simulink model "mpc_ttype_psm"  (R2026a)
settings: Solver=ode23tb  StopTime=param.sim.simlength  FixedStep=param.glb_time.tc  MaxStep=param.glb_time.tc
values from neighbouring files (symbols this model uses):
  param = struct()    [init_model.m]
libraries: fl_lib x25, nesl_utility x12, cstblocks_lti x6, lithium_ion_battery x1, dclink_for_three_levels x1, three_phase_three_level_ttype_inverter_ideal_switch_based_model x1, single_phase_pwm_modulator x1, threephase_inductor_lib x1, simple_flexible_shaft x1, permanent_magnet_synchronous_machine x1
(part 3 of 4)

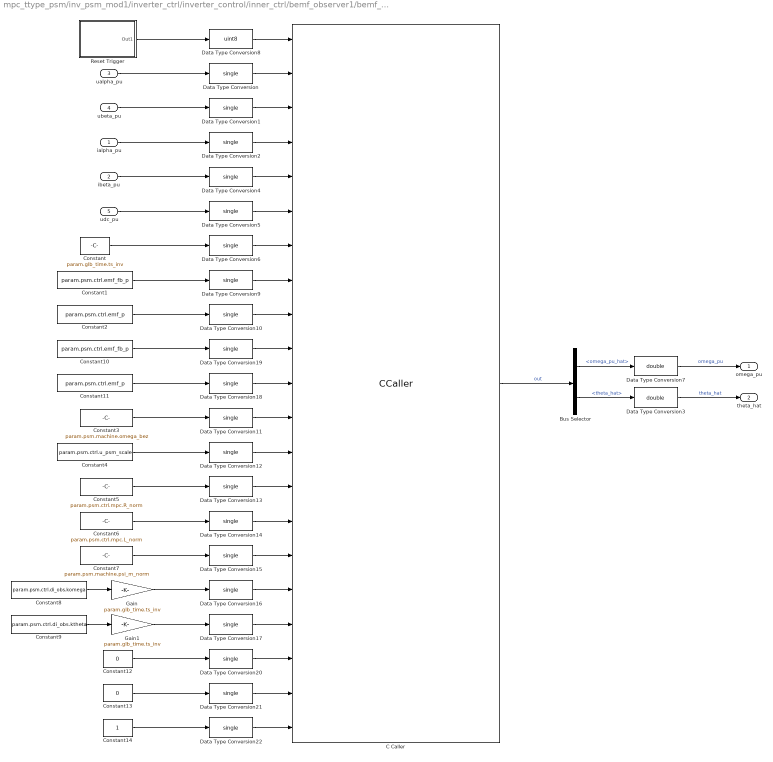
== system mpc_ttype_psm/inv_psm_mod1/inverter_ctrl/inverter_control/inner_ctrl/bemf_observer1/bemf_observer_ccaller ==
  ialpha_pu : Inport
  ibeta_pu : Inport  Port=2
  ualpha_pu : Inport  Port=3
  ubeta_pu : Inport  Port=4
  udc_pu : Inport  Port=5
  Bus Selector : BusSelector  OutputSignals=omega_pu_hat,theta_hat
  C Caller : CCaller  FunctionName=bemf_obsv_process_simulink  PortSpecificationStruct="%)30     .    N\"8   8    (     @         %    \"    !8    !     0         %  0 \"0    $    _    07)G3F%M90  4&]R=$YA;64 4V-O<&4     26YD97@     5'EP90      4VEZ90      27-';&]B86P   X    P    !@    @    $          4    (     0    ,    !         !   P!O=70 #@   #     &    \"     0         !0    @    !     P    $         $  # &]U=  .    .     8    (    !          %    \"     $    &     0         0  ...(+12985 chars)"
  Constant : Constant  Value=param.glb_time.ts_inv
  Constant1 : Constant  Value=param.psm.ctrl.emf_fb_p
  Constant10 : Constant  Value=param.psm.ctrl.emf_fb_p
  Constant11 : Constant  Value=param.psm.ctrl.emf_p
  Constant12 : Constant  Value=0
  Constant13 : Constant  Value=0
  Constant14 : Constant
  Constant2 : Constant  Value=param.psm.ctrl.emf_p
  Constant3 : Constant  Value=param.psm.machine.omega_bez
  Constant4 : Constant  Value=param.psm.ctrl.u_psm_scale
  Constant5 : Constant  Value=param.psm.ctrl.mpc.R_norm
  Constant6 : Constant  Value=param.psm.ctrl.mpc.L_norm
  Constant7 : Constant  Value=param.psm.machine.psi_m_norm
  Constant8 : Constant  Value=param.psm.ctrl.di_obs.komega
  Constant9 : Constant  Value=param.psm.ctrl.di_obs.ktheta
  Data Type Conversion{,1..2,4..6,9..22} (20 alike) : DataTypeConversion  OutDataTypeStr=single  SaturateOnIntegerOverflow=off  RndMeth=Floor
  Data Type Conversion3 : DataTypeConversion  OutDataTypeStr=double  SaturateOnIntegerOverflow=off  RndMeth=Floor
  Data Type Conversion7 : DataTypeConversion  OutDataTypeStr=double  SaturateOnIntegerOverflow=off  RndMeth=Floor
  Data Type Conversion8 : DataTypeConversion  OutDataTypeStr=uint8  SaturateOnIntegerOverflow=off  RndMeth=Floor
  Gain : Gain  Gain=param.glb_time.ts_inv
  Gain1 : Gain  Gain=param.glb_time.ts_inv
  Reset Trigger : Subsystem
  omega_pu : Outport
  theta_hat : Outport  Port=2
  wires:
  Data Type Conversion5/1 -> C Caller/6
  Data Type Conversion/1 -> C Caller/2
  C Caller/1 -> Bus Selector/1  "out"
  Data Type Conversion1/1 -> C Caller/3
  Data Type Conversion4/1 -> C Caller/5
  Data Type Conversion2/1 -> C Caller/4
  Data Type Conversion6/1 -> C Caller/7
  Bus Selector/2 -> Data Type Conversion3/1  "<theta_hat>"
  Bus Selector/1 -> Data Type Conversion7/1  "<omega_pu_hat>"
  Data Type Conversion7/1 -> omega_pu/1  "omega_pu"
  Data Type Conversion3/1 -> theta_hat/1  "theta_hat"
  Data Type Conversion8/1 -> C Caller/1
  Data Type Conversion9/1 -> C Caller/8
  Data Type Conversion10/1 -> C Caller/9
  Data Type Conversion19/1 -> C Caller/10
  Data Type Conversion18/1 -> C Caller/11
  Data Type Conversion11/1 -> C Caller/12
  Data Type Conversion12/1 -> C Caller/13
  Data Type Conversion13/1 -> C Caller/14
  Data Type Conversion14/1 -> C Caller/15
  Data Type Conversion15/1 -> C Caller/16
  Data Type Conversion16/1 -> C Caller/17
  Data Type Conversion17/1 -> C Caller/18
  Data Type Conversion20/1 -> C Caller/19
  Data Type Conversion21/1 -> C Caller/20
  Data Type Conversion22/1 -> C Caller/21
  Constant14/1 -> Data Type Conversion22/1
  Constant13/1 -> Data Type Conversion21/1
  Constant12/1 -> Data Type Conversion20/1
  Constant9/1 -> Gain1/1
  Constant8/1 -> Gain/1
  Constant7/1 -> Data Type Conversion15/1
  Constant6/1 -> Data Type Conversion14/1
  Constant5/1 -> Data Type Conversion13/1
  Constant4/1 -> Data Type Conversion12/1
  Constant3/1 -> Data Type Conversion11/1
  Constant11/1 -> Data Type Conversion18/1
  Constant10/1 -> Data Type Conversion19/1
  Constant2/1 -> Data Type Conversion10/1
  Constant1/1 -> Data Type Conversion9/1
  Constant/1 -> Data Type Conversion6/1
  ibeta_pu/1 -> Data Type Conversion4/1
  ialpha_pu/1 -> Data Type Conversion2/1
  ubeta_pu/1 -> Data Type Conversion1/1
  ualpha_pu/1 -> Data Type Conversion/1
  Reset Trigger/1(Out1) -> Data Type Conversion8/1
  udc_pu/1 -> Data Type Conversion5/1
  Gain/1 -> Data Type Conversion16/1
  Gain1/1 -> Data Type Conversion17/1

== system mpc_ttype_psm/inv_psm_mod1/inverter_ctrl/inverter_control/phase_compensation_1/alignment_ctrl/pi ==
  u_ref : Inport
  u : Inport  Port=2
  1/Ti : Gain  Gain=kp  SaturateOnIntegerOverflow=on  OutDataTypeStr=Inherit: Same as input  ParamDataTypeStr=Inherit: Same as input
  Saturation : Saturate  UpperLimit=lim_up  LowerLimit=lim_down
  Sum1 : Sum  Inputs=+++  SaturateOnIntegerOverflow=on
  Sum2 : Sum  Inputs=-+  SaturateOnIntegerOverflow=on
  Sum3 : Sum  Inputs=-+  SaturateOnIntegerOverflow=on
  Unit Delay4 : UnitDelay  SampleTime=-1
  kp : Gain  Gain=ki  SaturateOnIntegerOverflow=on  OutDataTypeStr=Inherit: Same as input  ParamDataTypeStr=Inherit: Same as input
  y : Outport
  wires:
  1/Ti/1 -> Sum1/1, Sum3/1
  kp/1 -> Sum1/2
  Sum3/1 -> Unit Delay4/1
  Unit Delay4/1 -> Sum1/3
  u_ref/1 -> Sum2/2
  u/1 -> Sum2/1
  Sum2/1 -> kp/1, 1/Ti/1
  Sum1/1 -> Saturation/1
  Saturation/1 -> Sum3/2, y/1

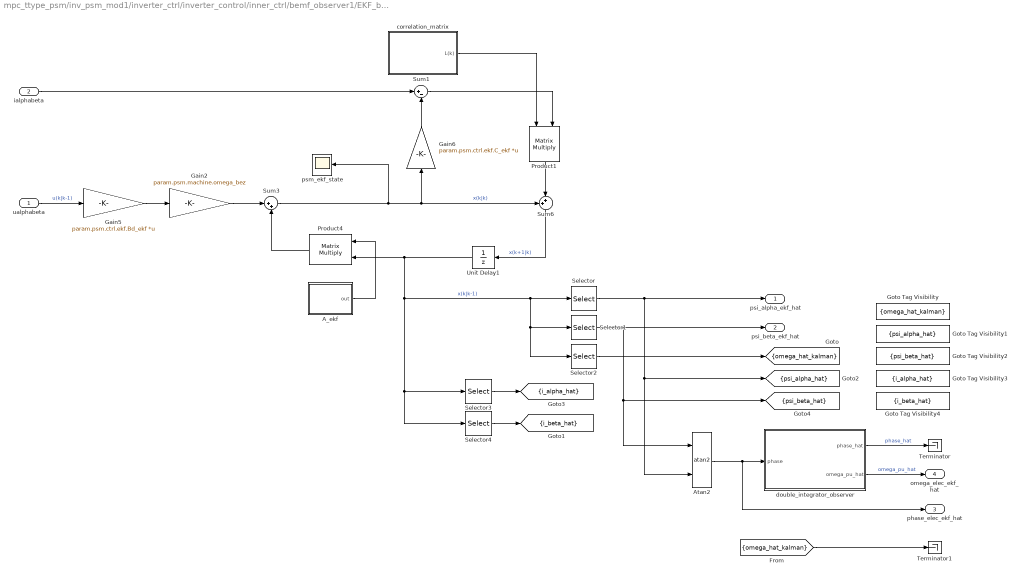
== system mpc_ttype_psm/inv_psm_mod1/inverter_ctrl/inverter_control/inner_ctrl/bemf_observer1/EKF_bemf_observer/extended_kalman_observer ==
  ualphabeta : Inport
  ialphabeta : Inport  Port=2
  A_ekf : Subsystem
  Atan2 : Trigonometry  Operator=atan2
  Gain2 : Gain  Gain=param.psm.machine.omega_bez
  Gain5 : Gain  Gain=param.psm.ctrl.ekf.Bd_ekf  Multiplication=Matrix(K*u)
  Gain6 : Gain  Gain=param.psm.ctrl.ekf.C_ekf  Multiplication=Matrix(K*u)
  Goto Tag Visibility : GotoTagVisibility  GotoTag=omega_hat_kalman
  Goto Tag Visibility1 : GotoTagVisibility  GotoTag=psi_alpha_hat
  Goto Tag Visibility2 : GotoTagVisibility  GotoTag=psi_beta_hat
  Goto Tag Visibility3 : GotoTagVisibility  GotoTag=i_alpha_hat
  Goto Tag Visibility4 : GotoTagVisibility  GotoTag=i_beta_hat
  Product1 : Product  Multiplication=Matrix(*)
  Product4 : Product  Multiplication=Matrix(*)
  Selector : Selector  InputPortWidth=6  IndexOptions=Index vector (dialog)  Indices=3  OutputSizes=1
  Selector1 : Selector  InputPortWidth=6  IndexOptions=Index vector (dialog)  Indices=4  OutputSizes=1
  Selector2 : Selector  InputPortWidth=6  IndexOptions=Index vector (dialog)  Indices=5  OutputSizes=1
  Selector3 : Selector  InputPortWidth=6  IndexOptions=Index vector (dialog)  Indices=1  OutputSizes=1
  Selector4 : Selector  InputPortWidth=6  IndexOptions=Index vector (dialog)  Indices=2  OutputSizes=1
  Sum1 : Sum  Inputs=|+-
  Sum3 : Sum  Inputs=|++
  Sum6 : Sum  Inputs=++|
  Terminator : Terminator
  Terminator1 : Terminator
  Unit Delay1 : UnitDelay  InitialCondition=[0 0 1 1 0 0]*param.glb_time.ts_inv  SampleTime=-1
  correlation_matrix : Subsystem
  double_integrator_observer : Subsystem
  psm_ekf_state : Scope
      settings: ActiveDisplayYMinimum=-3.1195074911927057  ActiveDisplayYMaximum=14.261541335565184
  psi_alpha_ekf_hat : Outport
  psi_beta_ekf_hat : Outport  Port=2
  phase_elec_ekf_hat : Outport  Port=3
  omega_elec_ekf_hat : Outport  Port=4
  tag scope: i_alpha_hat=scoped, i_beta_hat=scoped, omega_hat_kalman=scoped, psi_alpha_hat=scoped, psi_beta_hat=scoped
  wires:
  Gain5/1 -> Gain2/1
  Gain6/1 -> Sum1/2
  Sum6/1 -> Unit Delay1/1  "x(k+1|k)"
  Sum1/1 -> Product1/2
  ialphabeta/1 -> Sum1/1
  ualphabeta/1 -> Gain5/1  "u(k|k-1)"
  Sum3/1 -> psm_ekf_state/1, Gain6/1, Sum6/1  "x(k|k)"
  Unit Delay1/1 -> Selector2/1, Selector1/1, Selector/1, Selector3/1, Selector4/1, Product4/2  "x(k|k-1)"
  A_ekf/1(out) -> Product4/1
  Selector1/1 -> Atan2/1, [psi_beta_hat], psi_beta_ekf_hat/1
  Selector/1 -> Atan2/2, [psi_alpha_hat], psi_alpha_ekf_hat/1
  Selector2/1 -> [omega_hat_kalman]
  Selector3/1 -> [i_alpha_hat]
  Selector4/1 -> [i_beta_hat]
  Product4/1 -> Sum3/2
  Atan2/1 -> phase_elec_ekf_hat/1, double_integrator_observer/1(phase)
  Gain2/1 -> Sum3/1
  Product1/1 -> Sum6/2
  correlation_matrix/1(L(k)) -> Product1/1
  double_integrator_observer/1(phase_hat) -> Terminator/1  "phase_hat"
  double_integrator_observer/2(omega_pu_hat) -> omega_elec_ekf_hat/1  "omega_pu_hat"
  [omega_hat_kalman] -> Terminator1/1

== system mpc_ttype_psm/inv_psm_mod1/inverter_ctrl/inverter_control/inner_ctrl/bemf_observer1/bemf_observer/double_integrator_observer ==
  theta : Inport
  Dead Zone : DeadZone  LowerValue=-0.01  UpperValue=0.01
  Gain : Gain  Gain=param.psm.ctrl.di_obs.komega
  Gain1 : Gain  Gain=param.psm.ctrl.di_obs.ktheta
  Gain2 : Gain  Gain=param.psm.machine.omega_bez
  Gain3 : Gain  Gain=1/param.psm.machine.omega_bez
  Gain4 : Gain  Gain=param.glb_time.ts_inv
  Gain5 : Gain  Gain=param.glb_time.ts_inv
  Gain6 : Gain  Gain=param.glb_time.ts_inv
  Sum : Sum  Inputs=-+|
  Sum1 : Sum  Inputs=|++
  Sum2 : Sum  Inputs=|++
  Sum8 : Sum  Inputs=++|
  Unit Delay1 : UnitDelay  InitialCondition=pi  SampleTime=-1
  Unit Delay2 : UnitDelay  SampleTime=-1
  bounder1 : MATLAB Function  TreatAsAtomicUnit=on
  bounder2 : MATLAB Function  TreatAsAtomicUnit=on
  omega_pu_hat : Outport  VectorParamsAs1DForOutWhenUnconnected=off
  theta_hat : Outport  Port=2  VectorParamsAs1DForOutWhenUnconnected=off
  wires:
  Gain1/1 -> Gain6/1
  theta/1 -> Sum/2  "theta_bemf"
  Sum8/1 -> Unit Delay1/1
  Unit Delay1/1 -> bounder2/1(u)
  Sum1/1 -> Unit Delay2/1
  Gain/1 -> Gain4/1
  Unit Delay2/1 -> omega_pu_hat/1, Sum1/2, Gain5/1
  Sum2/1 -> Sum8/2
  bounder2/1(y) -> Sum2/2, theta_hat/1, Sum/1  "theta_hat"
  bounder1/1(y) -> Gain1/1, Gain/1
  Gain2/1 -> Sum8/1
  Gain3/1 -> Sum1/1
  Gain5/1 -> Gain2/1
  Sum/1 -> bounder1/1(u)
  Gain4/1 -> Gain3/1
  Gain6/1 -> Sum2/1

== system mpc_ttype_psm/inv_psm_mod1/inverter_ctrl/inverter_control/inner_ctrl/bemf_observer1/bemf_observer/psi_alpha_hat ==
  ualpha : Inport
  ialpha : Inport  Port=2
  udc : Inport  Port=3
  Gain1 : Gain  Gain=param.psm.ctrl.mpc.R_norm
  Gain2 : Gain  Gain=param.psm.ctrl.emf_fb_p
  Gain3 : Gain  Gain=param.psm.ctrl.emf_p
  Gain4 : Gain  Gain=param.psm.machine.omega_bez
  Gain5 : Gain  Gain=param.psm.ctrl.mpc.L_norm
  Gain6 : Gain  Gain=param.psm.ctrl.u_psm_scale
  Gain7 : Gain  Gain=param.glb_time.ts_inv
  Product : Product  RndMeth=Zero
  Sum : Sum  Inputs=|+-
  Sum1 : Sum  Inputs=|+-
  Sum2 : Sum  Inputs=++-  SaturateOnIntegerOverflow=on
  Sum3 : Sum  Inputs=|++
  Sum4 : Sum  Inputs=+-  SaturateOnIntegerOverflow=on
  Unit Delay1 : UnitDelay  SampleTime=-1
  Unit Delay2 : UnitDelay  SampleTime=-1
  Unit Delay3 : UnitDelay  SampleTime=-1
  psi_s_alpha_hat : Outport  VectorParamsAs1DForOutWhenUnconnected=off
  psi_r_alpha_hat : Outport  Port=2  VectorParamsAs1DForOutWhenUnconnected=off
  wires:
  [psi_r_m_alpha_mod1] -> Sum1/1
  [psi_r_alpha_hat_mod1] -> Sum1/2
  Gain4/1 -> Gain7/1
  Sum2/1 -> Gain4/1
  Gain3/1 -> Sum2/3
  ialpha/1 -> Gain5/1, Gain1/1
  Gain1/1 -> Sum/2
  Sum/1 -> Sum2/2
  ualpha/1 -> Product/1
  Gain5/1 -> Unit Delay3/1
  Unit Delay1/1 -> Sum4/1, psi_s_alpha_hat/1, Gain3/1, Sum3/2
  Sum3/1 -> Unit Delay1/1
  Sum4/1 -> Unit Delay2/1
  Sum1/1 -> Gain2/1
  Gain2/1 -> Sum2/1
  Gain7/1 -> Sum3/1
  Product/1 -> Gain6/1
  Gain6/1 -> Sum/1
  Unit Delay2/1 -> psi_r_alpha_hat/1
  Unit Delay3/1 -> Sum4/2
  udc/1 -> Product/2

== system mpc_ttype_psm/inv_psm_mod1/inverter_ctrl/inverter_control/inner_ctrl/bemf_observer1/bemf_observer/psi_beta_hat ==
  ubeta : Inport
  ibeta : Inport  Port=2
  udc : Inport  Port=3
  Gain1 : Gain  Gain=param.psm.ctrl.mpc.R_norm
  Gain2 : Gain  Gain=param.psm.ctrl.emf_fb_p
  Gain3 : Gain  Gain=param.psm.ctrl.emf_p
  Gain4 : Gain  Gain=param.psm.machine.omega_bez
  Gain5 : Gain  Gain=param.psm.ctrl.mpc.L_norm
  Gain6 : Gain  Gain=param.psm.ctrl.u_psm_scale
  Gain7 : Gain  Gain=param.glb_time.ts_inv
  Product : Product  RndMeth=Zero
  Sum : Sum  Inputs=|+-
  Sum1 : Sum  Inputs=|+-
  Sum2 : Sum  Inputs=++-  SaturateOnIntegerOverflow=on
  Sum3 : Sum  Inputs=|++
  Sum4 : Sum  Inputs=+-  SaturateOnIntegerOverflow=on
  Unit Delay1 : UnitDelay  SampleTime=-1
  Unit Delay2 : UnitDelay  SampleTime=-1
  Unit Delay3 : UnitDelay  SampleTime=-1
  psi_s_beta_hat : Outport  VectorParamsAs1DForOutWhenUnconnected=off
  psi_r_beta_hat : Outport  Port=2  VectorParamsAs1DForOutWhenUnconnected=off
  wires:
  Gain5/1 -> Unit Delay3/1
  Sum/1 -> Sum2/2
  Gain1/1 -> Sum/2
  ibeta/1 -> Gain5/1, Gain1/1
  Gain3/1 -> Sum2/3
  Sum2/1 -> Gain4/1
  Gain4/1 -> Gain7/1
  Sum1/1 -> Gain2/1
  [psi_r_beta_hat_mod1] -> Sum1/2
  [psi_r_m_beta_mod1] -> Sum1/1
  Unit Delay1/1 -> Gain3/1, Sum4/1, psi_s_beta_hat/1, Sum3/2
  Sum3/1 -> Unit Delay1/1
  Sum4/1 -> Unit Delay2/1
  Gain2/1 -> Sum2/1
  ubeta/1 -> Product/1
  Gain7/1 -> Sum3/1
  Product/1 -> Gain6/1
  Gain6/1 -> Sum/1
  Unit Delay2/1 -> psi_r_beta_hat/1
  Unit Delay3/1 -> Sum4/2
  udc/1 -> Product/2

== system mpc_ttype_psm/inv_psm_mod1/inverter_ctrl/inverter_control/inner_ctrl/bemf_observer1/bemf_observer/theta_bemf_hat ==
  psi_r_alpha_hat : Inport
  psi_r_beta_hat : Inport  Port=2
  Trigonometric Function : Trigonometry  Operator=atan2  OutputSignalType=real
  theta_emf_hat : Outport  VectorParamsAs1DForOutWhenUnconnected=off
  wires:
  psi_r_alpha_hat/1 -> Trigonometric Function/2
  psi_r_beta_hat/1 -> Trigonometric Function/1
  Trigonometric Function/1 -> theta_emf_hat/1

== system mpc_ttype_psm/inv_psm_mod1/inverter_ctrl/inverter_control/inner_ctrl/bemf_observer1/bemf_observer_ccaller/Reset Trigger ==
  Step : Step  Time=0.01  InitialValue=1  FinalValue=0
  Out1 : Outport
  wires:
  Step/1 -> Out1/1  "Reset"

== system mpc_ttype_psm/inv_psm_mod1/inverter_ctrl/inverter_control/inner_ctrl/bemf_observer1/EKF_bemf_observer/extended_kalman_observer/A_ekf ==
  Gain1 : Gain  Gain=param.psm.ctrl.ekf.A6_pred_ekf
  Gain{7,9..10,13,20} (5 alike) : Gain  Gain=param.psm.machine.omega_bez
  Gain{2,4,6,11,16,18} (6 alike) : Gain  Gain=param.glb_time.ts_inv
  Gain15 : Gain  Gain=param.psm.ctrl.ekf.A2_tilde_ekf
  Gain17 : Gain  Gain=param.psm.ctrl.ekf.A3_tilde_ekf
  Gain3 : Gain  Gain=param.psm.ctrl.ekf.A4_tilde_ekf
  Gain5 : Gain  Gain=param.psm.ctrl.ekf.A5_tilde_ekf
  I1 : Constant  Value=eye(6)
  I2 : Constant  Value=param.psm.ctrl.ekf.A1_tilde_ekf
  Sum7 : Sum  Inputs=+++++++
  out : Outport
  wires:
  Sum7/1 -> out/1
  I2/1 -> Gain11/1
  I1/1 -> Sum7/1
  Gain1/1 -> Gain2/1
  Gain3/1 -> Gain4/1
  Gain5/1 -> Gain6/1
  [omega_hat_kalman] -> Gain1/1
  [psi_alpha_hat] -> Gain3/1
  [psi_beta_hat] -> Gain5/1
  Gain11/1 -> Gain7/1
  Gain4/1 -> Gain9/1
  Gain6/1 -> Gain10/1
  Gain7/1 -> Sum7/2
  Gain9/1 -> Sum7/5
  Gain10/1 -> Sum7/6
  Gain18/1 -> Gain13/1
  Gain16/1 -> Gain20/1
  Gain17/1 -> Gain18/1
  Gain15/1 -> Gain16/1
  Gain13/1 -> Sum7/4
  Gain20/1 -> Sum7/3
  [i_beta_hat] -> Gain17/1
  [i_alpha_hat] -> Gain15/1
  Gain2/1 -> Sum7/7

== system mpc_ttype_psm/inv_psm_mod1/inverter_ctrl/inverter_control/inner_ctrl/bemf_observer1/EKF_bemf_observer/extended_kalman_observer/correlation_matrix ==
  A_ekf : Subsystem
  Gain1 : Gain  Gain=param.psm.ctrl.ekf.C_ekf  Multiplication=Matrix(u*K)
  Gain10 : Gain  Gain=param.psm.ctrl.ekf.C_ekf'  Multiplication=Matrix(u*K)
  Gain8 : Gain  Gain=param.psm.ctrl.ekf.C_ekf'  Multiplication=Matrix(u*K)
  Gain9 : Gain  Gain=param.psm.ctrl.ekf.C_ekf  Multiplication=Matrix(K*u)
  I6 : Constant  Value=eye(6)
  Product{,2,5..6} (4 alike) : Product  Multiplication=Matrix(*)
  Product3 : Product  Inputs=*/  Multiplication=Matrix(*)
  Q : Constant  Value=param.psm.ctrl.ekf.Qkalman
  R : Constant  Value=param.psm.ctrl.ekf.Rkalman
  R1 : Constant  Value=eye(2)
  Sum2 : Sum  Inputs=+-|
  Sum4 : Sum  Inputs=|++
  Sum5 : Sum  Inputs=|++
  Transpose : Math  Operator=transpose
  Unit Delay2 : UnitDelay  SampleTime=-1
  L(k) : Outport
  wires:
  A_ekf/1(out) -> Transpose/1, Product5/1
  Product6/1 -> Sum5/1
  Product3/1 -> Product/2
  Gain8/1 -> Product/1
  Sum4/1 -> Product3/2
  Sum5/1 -> Gain8/1, Gain9/1, Product2/2  "P(k|k)"
  Sum2/1 -> Product2/1
  Product/1 -> Gain1/1, L(k)/1  "L(k)"
  Gain1/1 -> Sum2/2
  R1/1 -> Product3/1
  Product2/1 -> Unit Delay2/1  "P(k+1|k)"
  Product5/1 -> Product6/1
  Gain10/1 -> Sum4/1
  Transpose/1 -> Product6/2
  R/1 -> Sum4/2
  Q/1 -> Sum5/2
  Unit Delay2/1 -> Product5/2
  Gain9/1 -> Gain10/1
  I6/1 -> Sum2/1

== system mpc_ttype_psm/inv_psm_mod1/inverter_ctrl/inverter_control/inner_ctrl/bemf_observer1/EKF_bemf_observer/extended_kalman_observer/double_integrator_observer ==
  phase : Inport
  Gain : Gain  Gain=param.psm.ctrl.di_obs.komega
  Gain1 : Gain  Gain=param.psm.ctrl.di_obs.ktheta
  Gain2 : Gain  Gain=param.psm.machine.omega_bez
  Gain3 : Gain  Gain=1/param.psm.machine.omega_bez
  Gain4 : Gain  Gain=param.glb_time.ts_inv
  Gain5 : Gain  Gain=param.glb_time.ts_inv
  Gain6 : Gain  Gain=param.glb_time.ts_inv
  Sum : Sum  Inputs=-+|
  Sum1 : Sum  Inputs=|++
  Sum2 : Sum  Inputs=|++
  Sum8 : Sum  Inputs=++|
  Unit Delay1 : UnitDelay  InitialCondition=pi  SampleTime=-1
  Unit Delay2 : UnitDelay  SampleTime=-1
  bounder1 : MATLAB Function  TreatAsAtomicUnit=on
  bounder2 : MATLAB Function  TreatAsAtomicUnit=on
  phase_hat : Outport  VectorParamsAs1DForOutWhenUnconnected=off
  omega_pu_hat : Outport  Port=2  VectorParamsAs1DForOutWhenUnconnected=off
  wires:
  Gain1/1 -> Gain6/1
  phase/1 -> Sum/2
  Sum8/1 -> Unit Delay1/1
  Unit Delay1/1 -> bounder2/1(u)
  Sum1/1 -> Unit Delay2/1
  Gain/1 -> Gain4/1
  Unit Delay2/1 -> omega_pu_hat/1, Sum1/2, Gain5/1
  Sum2/1 -> Sum8/2
  bounder2/1(y) -> Sum2/2, phase_hat/1, Sum/1  "phase_hat"
  bounder1/1(y) -> Gain/1, Gain1/1
  Gain2/1 -> Sum8/1
  Gain3/1 -> Sum1/1
  Gain5/1 -> Gain2/1
  Sum/1 -> bounder1/1(u)
  Gain4/1 -> Gain3/1
  Gain6/1 -> Sum2/1

== system mpc_ttype_psm/inv_psm_mod1/inverter_ctrl/inverter_control/inner_ctrl/bemf_observer1/EKF_bemf_observer/extended_kalman_observer/correlation_matrix/A_ekf ==
  Gain1 : Gain  Gain=param.psm.ctrl.ekf.A6_tilde_ekf
  Gain{7..10,13,20} (6 alike) : Gain  Gain=param.psm.machine.omega_bez
  Gain{2,4,6,11,16,18} (6 alike) : Gain  Gain=param.glb_time.ts_inv
  Gain15 : Gain  Gain=param.psm.ctrl.ekf.A2_tilde_ekf
  Gain17 : Gain  Gain=param.psm.ctrl.ekf.A3_tilde_ekf
  Gain3 : Gain  Gain=param.psm.ctrl.ekf.A4_tilde_ekf
  Gain5 : Gain  Gain=param.psm.ctrl.ekf.A5_tilde_ekf
  I1 : Constant  Value=eye(6)
  I2 : Constant  Value=param.psm.ctrl.ekf.A1_tilde_ekf
  Sum7 : Sum  Inputs=+++++++
  out : Outport
  wires:
  Sum7/1 -> out/1
  I2/1 -> Gain11/1
  I1/1 -> Sum7/1
  Gain1/1 -> Gain2/1
  Gain3/1 -> Gain4/1
  Gain5/1 -> Gain6/1
  [omega_hat_kalman] -> Gain1/1
  [psi_alpha_hat] -> Gain3/1
  [psi_beta_hat] -> Gain5/1
  Gain11/1 -> Gain7/1
  Gain2/1 -> Gain8/1
  Gain4/1 -> Gain9/1
  Gain6/1 -> Gain10/1
  Gain7/1 -> Sum7/2
  Gain9/1 -> Sum7/5
  Gain10/1 -> Sum7/6
  Gain8/1 -> Sum7/7
  Gain18/1 -> Gain13/1
  Gain16/1 -> Gain20/1
  Gain17/1 -> Gain18/1
  Gain15/1 -> Gain16/1
  Gain13/1 -> Sum7/4
  Gain20/1 -> Sum7/3
  [i_beta_hat] -> Gain17/1
  [i_alpha_hat] -> Gain15/1

== matlab function mpc_ttype_psm/inv_psm_mod1/inverter/deadtime_generator_for_ttype/dead_time_generator_cmos_simulink_phu/dead_time_leg_generator_1/MATLAB Function ==
  data: u input; y output; Vpos_rail_dtg parameter
function y = not_cmos(u, Vpos_rail_dtg)

vth = Vpos_rail_dtg/2;

if u > vth
    y = 0;
else
    y = Vpos_rail_dtg;
end

== matlab function mpc_ttype_psm/inv_psm_mod1/inverter/deadtime_generator_for_ttype/dead_time_generator_cmos_simulink_phu/dead_time_leg_generator_1/MATLAB Function1 ==
  data: u1 input; u2 input; y output; Vpos_rail_dtg parameter
function y = and_cmos(u1, u2, Vpos_rail_dtg)

vth = Vpos_rail_dtg/2;

if (u1 > vth && u2 > vth)
    y = Vpos_rail_dtg;
else
    y = 0;
end

== matlab function mpc_ttype_psm/inv_psm_mod1/inverter_ctrl/inverter_control/inner_ctrl/current_transformation/alphabeta2dq ==
  data: alpha input; d output; beta input; gamma input; q output
function [d,q] = alphabeta2dq(alpha,beta,gamma)

    d  =  alpha*cos(gamma) + beta*sin(gamma);
    q = -alpha*sin(gamma) + beta*cos(gamma);

end

== matlab function mpc_ttype_psm/inv_psm_mod1/inverter/deadtime_generator_for_ttype/dead_time_generator_cmos_simulink_phu/dead_time_leg_generator_1/MATLAB Function2 ==
  data: u input; y output; Vpos_rail_dtg parameter
function y = not_cmos(u, Vpos_rail_dtg)

vth = Vpos_rail_dtg/2;

if u > vth
    y = 0;
else
    y = Vpos_rail_dtg;
end

== matlab function mpc_ttype_psm/inv_psm_mod1/inverter/deadtime_generator_for_ttype/dead_time_generator_cmos_simulink_phu/dead_time_leg_generator_1/MATLAB Function3 ==
  data: u input; y output; Vpos_rail_dtg parameter
function y = not_cmos(u, Vpos_rail_dtg)

vth = Vpos_rail_dtg/2;

if u > vth
    y = 0;
else
    y = Vpos_rail_dtg;
end

== matlab function mpc_ttype_psm/inv_psm_mod1/inverter/deadtime_generator_for_ttype/dead_time_generator_cmos_simulink_phu/dead_time_leg_generator_1/MATLAB Function4 ==
  data: u1 input; u2 input; y output; Vpos_rail_dtg parameter
function y = and_cmos(u1, u2, Vpos_rail_dtg)

vth = Vpos_rail_dtg/2;

if (u1 > vth && u2 > vth)
    y = Vpos_rail_dtg;
else
    y = 0;
end

== matlab function mpc_ttype_psm/inv_psm_mod1/inverter_ctrl/inverter_control/inner_ctrl/current_transformation/uvw2alphabeta ==
  data: u input; alpha output; v input; w input; beta output
function [alpha,beta] = uvw2alphabeta(u,v,w)

alpha = 2/3*(u - 1/2*v - 1/2*w);
beta  = 2/3*(sqrt(3)/2*(v - w));

end

== matlab function mpc_ttype_psm/inv_psm_mod1/inverter/deadtime_generator_for_ttype/dead_time_generator_cmos_simulink_phu/dead_time_leg_generator_1/MATLAB Function5 ==
  data: u1 input; u2 input; y output; Vpos_rail_dtg parameter
function y = and_cmos(u1, u2, Vpos_rail_dtg)

vth = Vpos_rail_dtg/2;

if (u1 > vth && u2 > vth)
    y = Vpos_rail_dtg;
else
    y = 0;
end

== matlab function mpc_ttype_psm/inv_psm_mod1/inverter/deadtime_generator_for_ttype/dead_time_generator_cmos_simulink_phu/dead_time_leg_generator_1/MATLAB Function6 ==
  data: u input; y output; Vpos_rail_dtg parameter
function y = not_cmos(u, Vpos_rail_dtg)

vth = Vpos_rail_dtg/2;

if u > vth
    y = 0;
else
    y = Vpos_rail_dtg;
end

== matlab function mpc_ttype_psm/inv_psm_mod1/inverter/deadtime_generator_for_ttype/dead_time_generator_cmos_simulink_phu/dead_time_leg_generator_1/MATLAB Function7 ==
  data: u input; y output; Vpos_rail_dtg parameter
function y = not_cmos(u, Vpos_rail_dtg)

vth = Vpos_rail_dtg/2;

if u > vth
    y = 0;
else
    y = Vpos_rail_dtg;
end

== matlab function mpc_ttype_psm/inv_psm_mod1/inverter/deadtime_generator_for_ttype/dead_time_generator_cmos_simulink_phu/dead_time_leg_generator_1/MATLAB Function8 ==
  data: u input; y output; Vpos_rail_dtg parameter
function y = not_cmos(u, Vpos_rail_dtg)

vth = Vpos_rail_dtg/2;

if u > vth
    y = 0;
else
    y = Vpos_rail_dtg;
end

== matlab function mpc_ttype_psm/inv_psm_mod1/inverter/deadtime_generator_for_ttype/dead_time_generator_cmos_simulink_phu/dead_time_leg_generator_1/MATLAB Function9 ==
  data: u1 input; u2 input; y output; Vpos_rail_dtg parameter
function y = and_cmos(u1, u2, Vpos_rail_dtg)

vth = Vpos_rail_dtg/2;

if (u1 > vth && u2 > vth)
    y = Vpos_rail_dtg;
else
    y = 0;
end

== matlab function mpc_ttype_psm/inv_psm_mod1/inverter_ctrl/inverter_control/inner_ctrl/bemf_observer1/EKF_bemf_observer/extended_kalman_observer/double_integrator_observer/bounder2 ==
  data: u input; y output
function y = bounder(u)
    y = -pi + mod(u+3*pi,2*pi);
end

== matlab function mpc_ttype_psm/inv_psm_mod1/inverter_ctrl/inverter_control/inner_ctrl/bemf_observer1/bemf_observer/double_integrator_observer/bounder1 ==
  data: u input; y output
function y = bounder(u)
    
    y = -pi + mod(u+3*pi,2*pi);
end

== matlab function mpc_ttype_psm/inv_psm_mod1/inverter_ctrl/inverter_control/encoder-sensorless-switch/MATLAB Function ==
  data: omega_psm input; omega_ctrl output; phase_psm input; omega_obs input; phase_obs input; phase_ctrl output; omega_th input
function [omega_ctrl, phase_ctrl] = switch_enc2obs(omega_psm, phase_psm, omega_obs, phase_obs, omega_th)

if abs(omega_psm) > omega_th
    omega_ctrl = omega_obs;
    phase_ctrl = phase_obs;
else
    omega_ctrl = omega_psm;
    phase_ctrl = phase_psm;
end

== matlab function mpc_ttype_psm/inv_psm_mod1/inverter_ctrl/inverter_control/inner_ctrl/bemf_observer1/bemf_observer/double_integrator_observer/bounder2 ==
  data: u input; y output
function y = bounder(u)
    
    u = -pi + mod(u+3*pi,2*pi);
    
    y = u;
end

== matlab function mpc_ttype_psm/inv_psm_mod1/inverter/deadtime_generator_for_ttype/dead_time_generator_cmos_simulink_phv/dead_time_leg_generator_1/MATLAB Function ==
  data: u input; y output; Vpos_rail_dtg parameter
function y = not_cmos(u, Vpos_rail_dtg)

vth = Vpos_rail_dtg/2;

if u > vth
    y = 0;
else
    y = Vpos_rail_dtg;
end

== matlab function mpc_ttype_psm/inv_psm_mod1/inverter/deadtime_generator_for_ttype/dead_time_generator_cmos_simulink_phv/dead_time_leg_generator_1/MATLAB Function1 ==
  data: u1 input; u2 input; y output; Vpos_rail_dtg parameter
function y = and_cmos(u1, u2, Vpos_rail_dtg)

vth = Vpos_rail_dtg/2;

if (u1 > vth && u2 > vth)
    y = Vpos_rail_dtg;
else
    y = 0;
end

== matlab function mpc_ttype_psm/inv_psm_mod1/inverter/deadtime_generator_for_ttype/dead_time_generator_cmos_simulink_phv/dead_time_leg_generator_1/MATLAB Function2 ==
  data: u input; y output; Vpos_rail_dtg parameter
function y = not_cmos(u, Vpos_rail_dtg)

vth = Vpos_rail_dtg/2;

if u > vth
    y = 0;
else
    y = Vpos_rail_dtg;
end

== matlab function mpc_ttype_psm/inv_psm_mod1/inverter/deadtime_generator_for_ttype/dead_time_generator_cmos_simulink_phv/dead_time_leg_generator_1/MATLAB Function3 ==
  data: u input; y output; Vpos_rail_dtg parameter
function y = not_cmos(u, Vpos_rail_dtg)

vth = Vpos_rail_dtg/2;

if u > vth
    y = 0;
else
    y = Vpos_rail_dtg;
end

== matlab function mpc_ttype_psm/inv_psm_mod1/inverter/deadtime_generator_for_ttype/dead_time_generator_cmos_simulink_phv/dead_time_leg_generator_1/MATLAB Function4 ==
  data: u1 input; u2 input; y output; Vpos_rail_dtg parameter
function y = and_cmos(u1, u2, Vpos_rail_dtg)

vth = Vpos_rail_dtg/2;

if (u1 > vth && u2 > vth)
    y = Vpos_rail_dtg;
else
    y = 0;
end

== matlab function mpc_ttype_psm/inv_psm_mod1/inverter/deadtime_generator_for_ttype/dead_time_generator_cmos_simulink_phv/dead_time_leg_generator_1/MATLAB Function5 ==
  data: u1 input; u2 input; y output; Vpos_rail_dtg parameter
function y = and_cmos(u1, u2, Vpos_rail_dtg)

vth = Vpos_rail_dtg/2;

if (u1 > vth && u2 > vth)
    y = Vpos_rail_dtg;
else
    y = 0;
end

== matlab function mpc_ttype_psm/inv_psm_mod1/inverter/deadtime_generator_for_ttype/dead_time_generator_cmos_simulink_phv/dead_time_leg_generator_1/MATLAB Function6 ==
  data: u input; y output; Vpos_rail_dtg parameter
function y = not_cmos(u, Vpos_rail_dtg)

vth = Vpos_rail_dtg/2;

if u > vth
    y = 0;
else
    y = Vpos_rail_dtg;
end

== matlab function mpc_ttype_psm/inv_psm_mod1/inverter/deadtime_generator_for_ttype/dead_time_generator_cmos_simulink_phv/dead_time_leg_generator_1/MATLAB Function7 ==
  data: u input; y output; Vpos_rail_dtg parameter
function y = not_cmos(u, Vpos_rail_dtg)

vth = Vpos_rail_dtg/2;

if u > vth
    y = 0;
else
    y = Vpos_rail_dtg;
end

== matlab function mpc_ttype_psm/inv_psm_mod1/inverter/deadtime_generator_for_ttype/dead_time_generator_cmos_simulink_phv/dead_time_leg_generator_1/MATLAB Function8 ==
  data: u input; y output; Vpos_rail_dtg parameter
function y = not_cmos(u, Vpos_rail_dtg)

vth = Vpos_rail_dtg/2;

if u > vth
    y = 0;
else
    y = Vpos_rail_dtg;
end

== matlab function mpc_ttype_psm/inv_psm_mod1/inverter/deadtime_generator_for_ttype/dead_time_generator_cmos_simulink_phv/dead_time_leg_generator_1/MATLAB Function9 ==
  data: u1 input; u2 input; y output; Vpos_rail_dtg parameter
function y = and_cmos(u1, u2, Vpos_rail_dtg)

vth = Vpos_rail_dtg/2;

if (u1 > vth && u2 > vth)
    y = Vpos_rail_dtg;
else
    y = 0;
end

== matlab function mpc_ttype_psm/inv_psm_mod1/inverter/timer/MATLAB Function ==
  data: t input; y output; phase input; period input
function y = ramp_up_down(t,phase,period)
x = sin(2*pi/period*t - phase -pi/2);
y = asin(x)/pi + 1/2;

== matlab function mpc_ttype_psm/inv_psm_mod1/inverter/deadtime_generator_for_ttype/dead_time_generator_cmos_simulink_phw/dead_time_leg_generator_1/MATLAB Function ==
  data: u input; y output; Vpos_rail_dtg parameter
function y = not_cmos(u, Vpos_rail_dtg)

vth = Vpos_rail_dtg/2;

if u > vth
    y = 0;
else
    y = Vpos_rail_dtg;
end

== matlab function mpc_ttype_psm/inv_psm_mod1/inverter/deadtime_generator_for_ttype/dead_time_generator_cmos_simulink_phw/dead_time_leg_generator_1/MATLAB Function1 ==
  data: u1 input; u2 input; y output; Vpos_rail_dtg parameter
function y = and_cmos(u1, u2, Vpos_rail_dtg)

vth = Vpos_rail_dtg/2;

if (u1 > vth && u2 > vth)
    y = Vpos_rail_dtg;
else
    y = 0;
end

== matlab function mpc_ttype_psm/inv_psm_mod1/inverter/deadtime_generator_for_ttype/dead_time_generator_cmos_simulink_phw/dead_time_leg_generator_1/MATLAB Function2 ==
  data: u input; y output; Vpos_rail_dtg parameter
function y = not_cmos(u, Vpos_rail_dtg)

vth = Vpos_rail_dtg/2;

if u > vth
    y = 0;
else
    y = Vpos_rail_dtg;
end

== matlab function mpc_ttype_psm/inv_psm_mod1/inverter/deadtime_generator_for_ttype/dead_time_generator_cmos_simulink_phw/dead_time_leg_generator_1/MATLAB Function3 ==
  data: u input; y output; Vpos_rail_dtg parameter
function y = not_cmos(u, Vpos_rail_dtg)

vth = Vpos_rail_dtg/2;

if u > vth
    y = 0;
else
    y = Vpos_rail_dtg;
end

== matlab function mpc_ttype_psm/inv_psm_mod1/inverter/deadtime_generator_for_ttype/dead_time_generator_cmos_simulink_phw/dead_time_leg_generator_1/MATLAB Function4 ==
  data: u1 input; u2 input; y output; Vpos_rail_dtg parameter
function y = and_cmos(u1, u2, Vpos_rail_dtg)

vth = Vpos_rail_dtg/2;

if (u1 > vth && u2 > vth)
    y = Vpos_rail_dtg;
else
    y = 0;
end

== matlab function mpc_ttype_psm/inv_psm_mod1/inverter/deadtime_generator_for_ttype/dead_time_generator_cmos_simulink_phw/dead_time_leg_generator_1/MATLAB Function5 ==
  data: u1 input; u2 input; y output; Vpos_rail_dtg parameter
function y = and_cmos(u1, u2, Vpos_rail_dtg)

vth = Vpos_rail_dtg/2;

if (u1 > vth && u2 > vth)
    y = Vpos_rail_dtg;
else
    y = 0;
end

== matlab function mpc_ttype_psm/inv_psm_mod1/inverter/deadtime_generator_for_ttype/dead_time_generator_cmos_simulink_phw/dead_time_leg_generator_1/MATLAB Function6 ==
  data: u input; y output; Vpos_rail_dtg parameter
function y = not_cmos(u, Vpos_rail_dtg)

vth = Vpos_rail_dtg/2;

if u > vth
    y = 0;
else
    y = Vpos_rail_dtg;
end

== matlab function mpc_ttype_psm/inv_psm_mod1/inverter/deadtime_generator_for_ttype/dead_time_generator_cmos_simulink_phw/dead_time_leg_generator_1/MATLAB Function7 ==
  data: u input; y output; Vpos_rail_dtg parameter
function y = not_cmos(u, Vpos_rail_dtg)

vth = Vpos_rail_dtg/2;

if u > vth
    y = 0;
else
    y = Vpos_rail_dtg;
end

== matlab function mpc_ttype_psm/inv_psm_mod1/inverter/deadtime_generator_for_ttype/dead_time_generator_cmos_simulink_phw/dead_time_leg_generator_1/MATLAB Function8 ==
  data: u input; y output; Vpos_rail_dtg parameter
function y = not_cmos(u, Vpos_rail_dtg)

vth = Vpos_rail_dtg/2;

if u > vth
    y = 0;
else
    y = Vpos_rail_dtg;
end

== matlab function mpc_ttype_psm/inv_psm_mod1/inverter/deadtime_generator_for_ttype/dead_time_generator_cmos_simulink_phw/dead_time_leg_generator_1/MATLAB Function9 ==
  data: u1 input; u2 input; y output; Vpos_rail_dtg parameter
function y = and_cmos(u1, u2, Vpos_rail_dtg)

vth = Vpos_rail_dtg/2;

if (u1 > vth && u2 > vth)
    y = Vpos_rail_dtg;
else
    y = 0;
end

== matlab function mpc_ttype_psm/inv_psm_mod1/inverter_ctrl/inverter_control/encoder-sensorless-switch/double_integrator_observer/bounder1 ==
  data: u input; y output
function y = bounder(u)
    y = -pi + mod(u+3*pi,2*pi);
end

== matlab function mpc_ttype_psm/inv_psm_mod1/inverter_ctrl/inverter_control/encoder-sensorless-switch/double_integrator_observer/bounder2 ==
  data: u input; y output
function y = bounder(u)
    y = -pi + mod(u+3*pi,2*pi);
end

== matlab function mpc_ttype_psm/inv_psm_mod1/inverter_ctrl/inverter_control/inner_ctrl/bemf_observer1/EKF_bemf_observer/extended_kalman_observer/double_integrator_observer/bounder1 ==
  data: u input; y output
function y = bounder(u)
    y = -pi + mod(u+3*pi,2*pi);
end
